simulink model "simrt_workflow_probe"  (R2024b)
settings: Solver=FixedStepDiscrete  StartTime=0.0  StopTime=inf  FixedStep=0.001  RelTol=1e-3
model workspace (MAT data in the model file):
  CalGain = Simulink.Parameter
  CalGain.Value = 2
  CalGain.Complexity = 'real'
  CalGain.Dimensions = [1 1]
  CalGain.DataType = 'auto'
  CalGain.Min = 0
  CalGain.Max = 20
  CalOffset = Simulink.Parameter
  CalOffset.Value = 0
  CalOffset.Complexity = 'real'
  CalOffset.Dimensions = [1 1]
  CalOffset.DataType = 'auto'
  CalOffset.Min = -10
  CalOffset.Max = 10
  InputAmplitude = Simulink.Parameter
  InputAmplitude.Value = 1
  InputAmplitude.Complexity = 'real'
  InputAmplitude.Dimensions = [1 1]
  InputAmplitude.DataType = 'auto'
  InputAmplitude.Min = 0
  InputAmplitude.Max = 10
  OutputLowerLimit = Simulink.Parameter
  OutputLowerLimit.Value = -10
  OutputLowerLimit.Complexity = 'real'
  OutputLowerLimit.Dimensions = [1 1]
  OutputLowerLimit.DataType = 'auto'
  OutputLowerLimit.Min = -100
  OutputLowerLimit.Max = 0
  OutputUpperLimit = Simulink.Parameter
  OutputUpperLimit.Value = 10
  OutputUpperLimit.Complexity = 'real'
  OutputUpperLimit.Dimensions = [1 1]
  OutputUpperLimit.DataType = 'auto'
  OutputUpperLimit.Min = 0
  OutputUpperLimit.Max = 100
settings Model: Creator=yonggang.zhang  LastModifiedBy=yonggang.zhang
settings OptimizationCC: EnhancedBackFolding=on  PassReuseOutputArgsAs=Individual arguments  ZeroExternalMemoryAtStartup=off  ZeroInternalMemoryAtStartup=off  MaxStackSize=64  OptimizeBlockOrder=speed  DifferentSizesBufferReuse=on  OptimizationCustomize=off  EfficientTunableParamExpr=on
settings DebuggingCC: ParameterTunabilityLossMsg=error
settings HardwareCC: ProdBitPerLong=64  ProdHWDeviceType=Intel->x86-64 (Linux 64)
settings SFSimCC: MATLABDynamicMemAlloc=off
settings RTWCC: Description=Embedded Coder  SystemTargetFile=ert.tlc  HardwareBoard=SimRT  TLCOptions="-aInlineSetEventsForThisBaseRateFcn=TLC_FALSE -aSuppressMultiTaskScheduler=TLC_FALSE  -aRateBasedStepFcn=0"  TemplateMakefile=ert_default_tmf  Toolchain=SimRT portable-linux-toolchain
settings CodeAppCC: ForceParamTrailComments=on  IgnoreCustomStorageClasses=off  OperatorAnnotations=on  SimulinkDataObjDesc=on  SFDataObjDesc=on  InsertBlockDesc=on
settings ERTTargetCC: ExtMode=on  ExtModeTransport=2  ExtModeStaticAlloc=on  ExtModeMexFile=ext_xcp  ExtModeIntrfLevel=Level2 - Open  InlinedParameterPlacement=Hierarchical

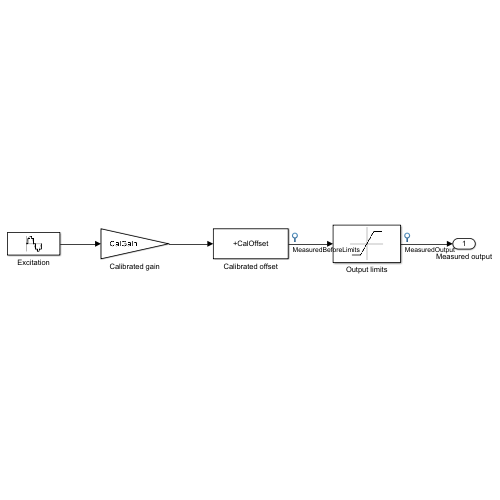
[thumbnail: Simulink's stored preview of the top-level diagram]
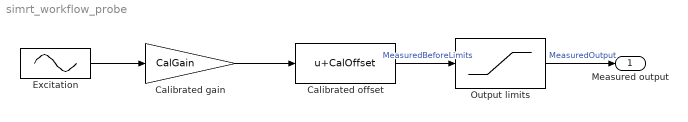
== system simrt_workflow_probe ==
  Calibrated gain : Gain  Gain=CalGain
  Calibrated offset : Bias  Bias=CalOffset  SaturateOnIntegerOverflow=off
  Excitation : Sin  Amplitude=InputAmplitude  SampleTime=0.001
  Output limits : Saturate  UpperLimit=OutputUpperLimit  LowerLimit=OutputLowerLimit
  Measured output : Outport
  wires:
  Excitation/1 -> Calibrated gain/1
  Calibrated gain/1 -> Calibrated offset/1
  Calibrated offset/1 -> Output limits/1  "MeasuredBeforeLimits"
  Output limits/1 -> Measured output/1  "MeasuredOutput"
